simulink model "part1_daily_profiles"  (R2026a)
settings: Solver=ode1  StopTime=24.0  FixedStep=0.01
libraries: simulink x5
settings Model: Creator=HAKAN SARI  LastModifiedBy=HAKAN SARI

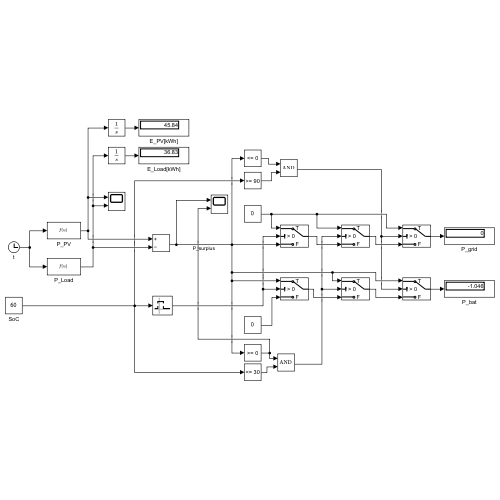
[thumbnail: Simulink's stored preview of the top-level diagram]
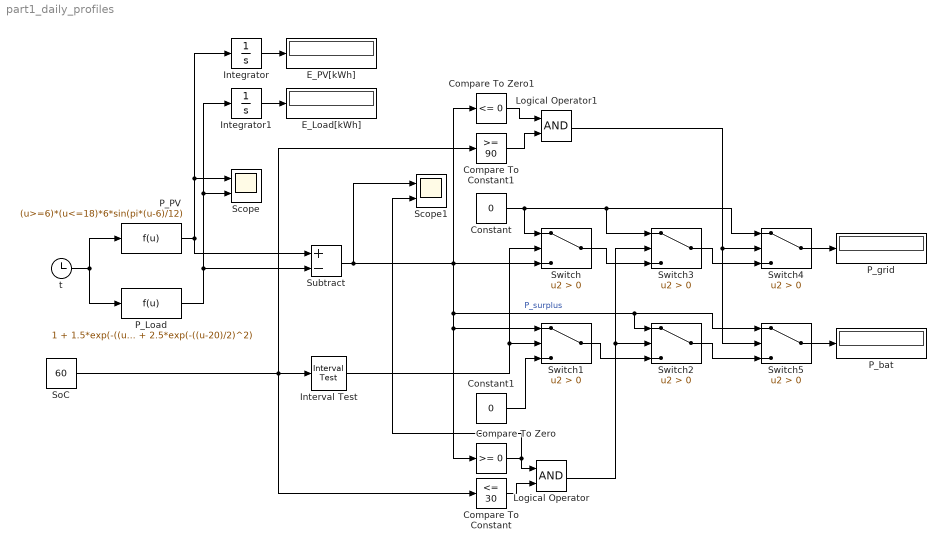
== system part1_daily_profiles ==
  Compare To Constant : simulink/Logic and Bit Operations/Compare To Constant  relop=<=  const=30  OutDataTypeStr=boolean
  Compare To Constant1 : simulink/Logic and Bit Operations/Compare To Constant  relop=>=  const=90  OutDataTypeStr=boolean
  Compare To Zero : simulink/Logic and Bit Operations/Compare To Zero  relop=>=  OutDataTypeStr=boolean
  Compare To Zero1 : simulink/Logic and Bit Operations/Compare To Zero  relop=<=  OutDataTypeStr=boolean
  Constant : Constant  Value=0
  Constant1 : Constant  Value=0
  E_Load[kWh] : Display
  E_PV[kWh] : Display
  Integrator : Integrator
  Integrator1 : Integrator
  Interval Test : simulink/Logic and Bit Operations/Interval Test  IntervalClosedRight=off  uplimit=90  IntervalClosedLeft=off  lowlimit=30  OutDataTypeStr=boolean
  Logical Operator : Logic  AllPortsSameDT=off  OutDataTypeStr=boolean
  Logical Operator1 : Logic  AllPortsSameDT=off  OutDataTypeStr=boolean
  P_Load : Fcn  Expr=1 + 1.5*exp(-((u-8)/1.5)^2) + 2.5*exp(-((u-20)/2)^2)
  P_PV : Fcn  Expr=(u>=6)*(u<=18)*6*sin(pi*(u-6)/12)
  P_bat : Display
  P_grid : Display
  Scope : Scope  NumInputPorts=2
      settings: ActiveDisplayYMinimum=-1  ActiveDisplayYMaximum=1
  Scope1 : Scope  NumInputPorts=2
      settings: ActiveDisplayYMinimum=-1  ActiveDisplayYMaximum=1
  SoC : Constant  Value=60
  Subtract : Sum  Inputs=+-
  Switch{,1..5} (6 alike) : Switch  Criteria=u2 > Threshold  SaturateOnIntegerOverflow=off  InputSameDT=off
  t : Clock
  wires:
  P_PV/1 -> Integrator/1, Scope/1, Subtract/1
  P_Load/1 -> Integrator1/1, Scope/2, Subtract/2
  Subtract/1 -> Switch5/1, Switch2/1, Compare To Zero/1, Switch1/1, Compare To Zero1/1, Switch/3, Scope1/1  "P_surplus"
  SoC/1 -> Interval Test/1, Compare To Constant/1, Compare To Constant1/1
  Interval Test/1 -> Switch1/2, Switch/2
  Constant/1 -> Switch4/1, Switch3/1, Switch/1
  Constant1/1 -> Switch1/3
  Compare To Constant/1 -> Logical Operator/2
  Compare To Zero/1 -> Scope1/2, Logical Operator/1
  Logical Operator/1 -> Switch3/2, Switch2/2
  Switch1/1 -> Switch2/3
  Compare To Zero1/1 -> Logical Operator1/1
  Compare To Constant1/1 -> Logical Operator1/2
  Switch/1 -> Switch3/3
  Switch4/1 -> P_grid/1
  Switch5/1 -> P_bat/1
  Logical Operator1/1 -> Switch5/2, Switch4/2
  Switch3/1 -> Switch4/3
  Switch2/1 -> Switch5/3
  t/1 -> P_PV/1, P_Load/1
  Integrator/1 -> E_PV[kWh]/1
  Integrator1/1 -> E_Load[kWh]/1
